simulink model "Mdl_qLPV_5states"  (R2023a)
settings: Solver=FixedStepAuto  StartTime=0.0  StopTime=10.0  FixedStep=DT  RelTol=1e-3
values from neighbouring files (symbols this model uses):
  beta = 0.0 0.0017453292519943296 0.0034906585039886592 0.005235987755982989 0.0069813170079773184 0.0087266462599716477 0.010471975511965978 0.012217304763960306 0.013962634015954637 0.015707963267948967 0.017453292519943295 0.019198621771937627 0.020943951023931956 0.022689280275926284 0.024434609527920613 0.026179938779914941 0.027925268031909273 0.029670597283903605 0.031415926535897934 0.033161255787    [DD_Mdl1.sldd]
  Cq = 0.0 0.0 0.0 0.0 0.0 0.0 0.0 0.0 0.0 0.0 0.0 0.0 0.0 0.0 0.0 0.0 0.0 0.0 0.0 0.0 0.0 0.0 0.0 0.0 0.0 0.0 0.0 0.0 0.0 0.0 0.0 0.0 0.0 0.0 0.0 0.0 0.0 0.0 0.0 0.0 0.0 0.0 0.0 0.0 0.0 0.0 0.0 0.0 0.0 0.0 0.0 0.0 0.0 0.0 0.0 0.0 0.0 0.0 0.0 0.0 0.0 0.0 0.0 0.0 0.0 0.0 0.0 0.0 0.0 0.0 0.0 0.0 0.0 0.0 0.0 0.0 0.0 0.0 0.0 0.0 0.0 0.0 0.0 0.0 0.0 0.0 0.0 0.0 0.0 0.0 0.0 0.0 0.0 0.0 0.0 0.0 0.0 0.0 0.0 0.0    [DD_Mdl1.sldd]
  Ct = 0.0 0.0 0.0 0.0 0.0 0.0 0.0 0.0 0.0 0.0 0.0 0.0 0.0 0.0 0.0 0.0 0.0 0.0 0.0 0.0 0.0 0.0 0.0 0.0 0.0 0.0 0.0 0.0 0.0 0.0 0.0 0.0 0.0 0.0 0.0 0.0 0.0 0.0 0.0 0.0 0.0 0.0 0.0 0.0 0.0 0.0 0.0 0.0 0.0 0.0 0.0 0.0 0.0 0.0 0.0 0.0 0.0 0.0 0.0 0.0 0.0 0.0 0.0 0.0 0.0 0.0 0.0 0.0 0.0 0.0 0.0 0.0 0.0 0.0 0.0 0.0 0.0 0.0 0.0 0.0 0.0 0.0 0.0 0.0 0.0 0.0 0.0 0.0 0.0 0.0 0.0 0.0 0.0 0.0 0.0 0.0 0.0 0.0 0.0 0.0    [DD_Mdl1.sldd]
  lambda = 0.0 0.1 0.2 0.30000000000000004 0.4 0.5 0.60000000000000009 0.70000000000000007 0.8 0.9 1.0 1.1 1.2000000000000002 1.3 1.4000000000000001 1.5 1.6 1.7000000000000002 1.8 1.9000000000000001 2.0 2.1 2.2 2.3000000000000003 2.4000000000000004 2.5 2.6 2.7 2.8000000000000003 2.9000000000000004 3.0 3.1 3.2 3.3000000000000003 3.4000000000000004 3.5 3.6 3.7 3.8000000000000003 3.9000000000000004 4.0 4.100000    [DD_Mdl1.sldd]
  rho = 1.225    [DD_Mdl1.sldd]
  wecs = 3.0    [DD_Mdl1.sldd]    (also in wecsmatfile.m = struct)
settings Model: DataDictionary=DD_Mdl1.sldd  Creator=ditt_aj  LastModifiedBy=ditt_aj
settings SolverCC: AlgebraicLoopSolver=TrustRegion
settings DebuggingCC: UnconnectedInputMsg=warning  UnconnectedOutputMsg=warning  UnconnectedLineMsg=warning
settings ModelReferenceCC: EnableRefExpFcnMdlSchedulingChecks=on
settings SFSimCC: CustomCodeUndefinedFunction=UseInterfaceOnly
settings RTWCC: DLArmComputeVersion=19.05

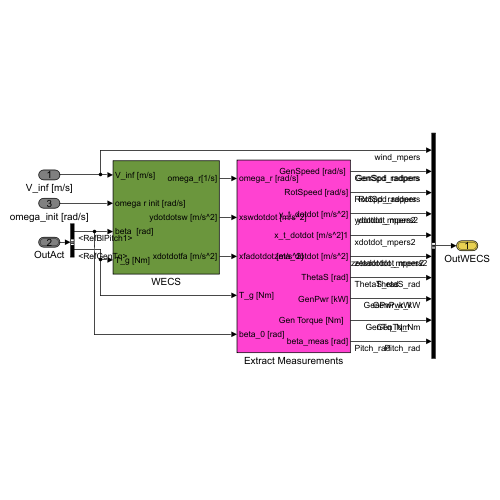
[thumbnail: Simulink's stored preview of the top-level diagram]
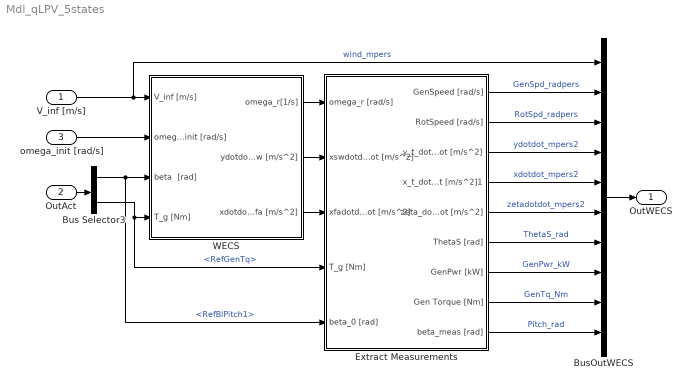
== system Mdl_qLPV_5states ==
  V_inf [m/s] : Inport
  OutAct : Inport  Port=2  OutDataTypeStr=Bus: slBus2
  omega_init [rad/s] : Inport  Port=3
  Bus Selector3 : BusSelector  OutputSignals=RefBlPitch1,RefGenTq
  BusOutWECS : BusCreator  Inputs=10  OutDataTypeStr=Bus: slBus1
  Extract Measurements : Subsystem
  WECS : Subsystem
  OutWECS : Outport  OutDataTypeStr=Bus: slBus1
  wires:
  Bus Selector3/2 -> Extract Measurements/4(T_g [Nm]), WECS/4(T_g [Nm])  "<RefGenTq>"
  Bus Selector3/1 -> Extract Measurements/5(beta_0 [rad]), WECS/3(beta  [rad])  "<RefBlPitch1>"
  V_inf [m/s]/1 -> BusOutWECS/1, WECS/1(V_inf [m/s])  "wind_mpers"
  omega_init [rad/s]/1 -> WECS/2(omega r init [rad/s])
  WECS/2(ydotdotsw [m/s^2]) -> Extract Measurements/2(xswdotdot [m/s^2])
  WECS/3(xdotdotfa [m/s^2]) -> Extract Measurements/3(xfadotdot [m/s^2])
  WECS/1(omega_r[1/s]) -> Extract Measurements/1("omega_r [rad/s] ")
  Extract Measurements/5(zeta_dotdot [m/s^2]) -> BusOutWECS/6  "zetadotdot_mpers2"
  Extract Measurements/4(x_t_dotdot [m/s^2]1) -> BusOutWECS/5  "xdotdot_mpers2"
  Extract Measurements/2(" RotSpeed [rad/s]") -> BusOutWECS/3  "RotSpd_radpers"
  Extract Measurements/3(y_t_dotdot [m/s^2]) -> BusOutWECS/4  "ydotdot_mpers2"
  Extract Measurements/8("Gen Torque [Nm]  ") -> BusOutWECS/9  "GenTq_Nm"
  Extract Measurements/6(ThetaS [rad]) -> BusOutWECS/7  "ThetaS_rad"
  Extract Measurements/1("GenSpeed [rad/s] ") -> BusOutWECS/2  "GenSpd_radpers"
  Extract Measurements/9(beta_meas [rad]) -> BusOutWECS/10  "Pitch_rad"
  Extract Measurements/7(GenPwr [kW]) -> BusOutWECS/8  "GenPwr_kW"
  BusOutWECS/1 -> OutWECS/1
  OutAct/1 -> Bus Selector3/1

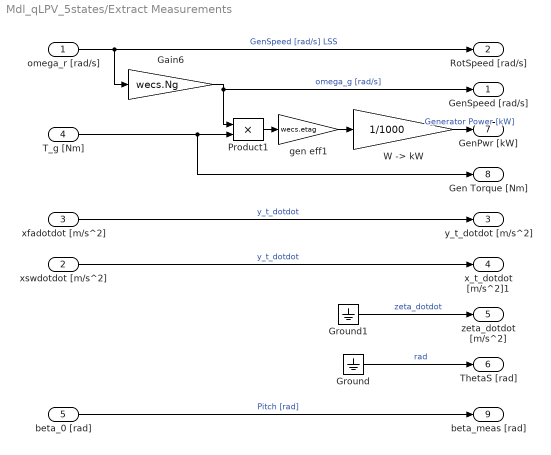
== system Mdl_qLPV_5states/Extract Measurements ==
  "omega_r [rad/s] " : Inport
  xswdotdot [m/s^2] : Inport  Port=2
  xfadotdot [m/s^2] : Inport  Port=3
  T_g [Nm] : Inport  Port=4
  beta_0 [rad] : Inport  Port=5
  Gain6 : Gain  Gain=wecs.Ng
  Ground : Ground
  Ground1 : Ground
  Product1 : Product  RndMeth=Zero
  "W -> kW" : Gain  Gain=1/1000
  gen eff1 : Gain  Gain=wecs.etag
  "GenSpeed [rad/s] " : Outport  VectorParamsAs1DForOutWhenUnconnected=off
  " RotSpeed [rad/s]" : Outport  Port=2  VectorParamsAs1DForOutWhenUnconnected=off
  y_t_dotdot [m/s^2] : Outport  Port=3  VectorParamsAs1DForOutWhenUnconnected=off
  x_t_dotdot [m/s^2]1 : Outport  Port=4  VectorParamsAs1DForOutWhenUnconnected=off
  zeta_dotdot [m/s^2] : Outport  Port=5  VectorParamsAs1DForOutWhenUnconnected=off
  ThetaS [rad] : Outport  Port=6  VectorParamsAs1DForOutWhenUnconnected=off
  GenPwr [kW] : Outport  Port=7  VectorParamsAs1DForOutWhenUnconnected=off
  "Gen Torque [Nm]  " : Outport  Port=8  VectorParamsAs1DForOutWhenUnconnected=off
  beta_meas [rad] : Outport  Port=9  VectorParamsAs1DForOutWhenUnconnected=off
  wires:
  xfadotdot [m/s^2]/1 -> y_t_dotdot [m/s^2]/1  "y_t_dotdot"
  Gain6/1 -> "GenSpeed [rad/s] "/1, Product1/1  "omega_g [rad/s]"
  T_g [Nm]/1 -> "Gen Torque [Nm]  "/1, Product1/2
  Ground/1 -> ThetaS [rad]/1  "rad"
  "omega_r [rad/s] "/1 -> " RotSpeed [rad/s]"/1, Gain6/1  "GenSpeed [rad/s] LSS"
  Product1/1 -> gen eff1/1
  Ground1/1 -> zeta_dotdot [m/s^2]/1  "zeta_dotdot"
  gen eff1/1 -> "W -> kW"/1
  "W -> kW"/1 -> GenPwr [kW]/1  "Generator Power [kW]"
  xswdotdot [m/s^2]/1 -> x_t_dotdot [m/s^2]1/1  "y_t_dotdot"
  beta_0 [rad]/1 -> beta_meas [rad]/1  "Pitch [rad]"

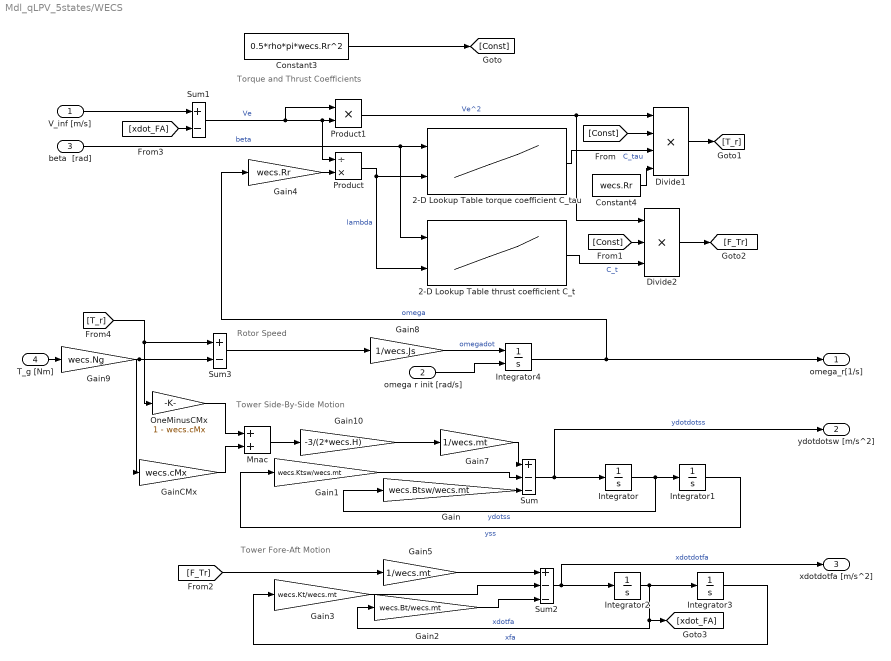
== system Mdl_qLPV_5states/WECS ==
  note: Tower Fore-Aft Motion
  note: Rotor Speed
  note: Torque and Thrust Coefficients
  note: Tower Side-By-Side Motion
  V_inf [m/s] : Inport
  omega r init [rad/s] : Inport  Port=2
  beta  [rad] : Inport  Port=3
  T_g [Nm] : Inport  Port=4
  2-D Lookup Table thrust coefficient C_t : Lookup_n-D  BreakpointsForDimension1=beta  BreakpointsForDimension2=lambda  Table=Ct  InterpMethod=Cubic spline  InternalRulePriority=Speed  RndMeth=Simplest
      settings: InputPortMap=u0,u1
  2-D Lookup Table torque coefficient C_tau : Lookup_n-D  BreakpointsForDimension1=beta  BreakpointsForDimension2=lambda  Table=Cq  InterpMethod=Cubic spline  InternalRulePriority=Speed  RndMeth=Simplest
      settings: InputPortMap=u0,u1
  Constant3 : Constant  Value=0.5*rho*pi*wecs.Rr^2
  Constant4 : Constant  Value=wecs.Rr
  Divide1 : Product  Inputs=****
  Divide2 : Product  Inputs=***
  Gain : Gain  Gain=wecs.Btsw/wecs.mt
  Gain1 : Gain  Gain=wecs.Ktsw/wecs.mt
  Gain10 : Gain  Gain=-3/(2*wecs.H)
  Gain2 : Gain  Gain=wecs.Bt/wecs.mt
  Gain3 : Gain  Gain=wecs.Kt/wecs.mt
  Gain4 : Gain  Gain=wecs.Rr
  Gain5 : Gain  Gain=1/wecs.mt
  Gain7 : Gain  Gain=1/wecs.mt
  Gain8 : Gain  Gain=1/wecs.Js
  Gain9 : Gain  Gain=wecs.Ng
  GainCMx : Gain  Gain=wecs.cMx
  Integrator{,1..3} (4 alike) : Integrator
  Integrator4 : Integrator  InitialConditionSource=external  InitialCondition=0.7853
  Mnac : Sum  Description=Torsional nacelle moment M_x = (1 - cMx)*Tr + cMx*Ng*Tg
  OneMinusCMx : Gain  Gain=1 - wecs.cMx
  Product : Product  Inputs=/*
  Product1 : Product  Inputs=**
  Sum : Sum  Inputs=+--
  Sum1 : Sum  Inputs=+-
  Sum2 : Sum  Inputs=+--
  Sum3 : Sum  Inputs=+-
  omega_r[1/s] : Outport  VectorParamsAs1DForOutWhenUnconnected=off
  ydotdotsw [m/s^2] : Outport  Port=2  VectorParamsAs1DForOutWhenUnconnected=off
  xdotdotfa [m/s^2] : Outport  Port=3  VectorParamsAs1DForOutWhenUnconnected=off
  wires:
  Product1/1 -> Divide1/1, Divide2/1  "Ve^2"
  Integrator2/1 -> Integrator3/1, [xdot_FA], Gain2/1  "xdotfa"
  Sum2/1 -> Integrator2/1, xdotdotfa [m/s^2]/1  "xdotdotfa"
  Integrator4/1 -> omega_r[1/s]/1, Gain4/1  "omega"
  Constant3/1 -> [Const]
  Gain5/1 -> Sum2/1
  Product/1 -> 2-D Lookup Table thrust coefficient C_t/2, 2-D Lookup Table torque coefficient C_tau/2  "lambda"
  Constant4/1 -> Divide1/4
  Sum1/1 -> Product1/1, Product1/2, Product/1  "Ve"
  Gain2/1 -> Sum2/3
  Integrator3/1 -> Gain3/1  "xfa"
  Gain3/1 -> Sum2/2
  Gain4/1 -> Product/2
  [T_r] -> OneMinusCMx/1, Sum3/1
  beta  [rad]/1 -> 2-D Lookup Table thrust coefficient C_t/1, 2-D Lookup Table torque coefficient C_tau/1  "beta"
  Divide2/1 -> [F_Tr]
  2-D Lookup Table thrust coefficient C_t/1 -> Divide2/3  "C_t"
  Gain9/1 -> GainCMx/1, Sum3/2
  Gain8/1 -> Integrator4/1  "omegadot"
  Divide1/1 -> [T_r]
  [Const] -> Divide1/2
  [Const] -> Divide2/2
  2-D Lookup Table torque coefficient C_tau/1 -> Divide1/3  "C_tau"
  [F_Tr] -> Gain5/1
  Gain/1 -> Sum/3
  Sum/1 -> Integrator/1, ydotdotsw [m/s^2]/1  "ydotdotss"
  Gain1/1 -> Sum/2
  Gain7/1 -> Sum/1
  Integrator/1 -> Integrator1/1, Gain/1  "ydotss"
  T_g [Nm]/1 -> Gain9/1
  Integrator1/1 -> Gain1/1  "yss"
  Gain10/1 -> Gain7/1
  omega r init [rad/s]/1 -> Integrator4/2
  Sum3/1 -> Gain8/1
  GainCMx/1 -> Mnac/2
  Mnac/1 -> Gain10/1
  OneMinusCMx/1 -> Mnac/1
  V_inf [m/s]/1 -> Sum1/1
  [xdot_FA] -> Sum1/2
